simulink model "DPC_POWER_RAHMAN_original(1)"  (R2022a)
settings: Solver=VariableStepAuto  StartTime=0.0  StopTime=10  FixedStep=Ts  RelTol=1e-3
undefined symbols (not defined in the file): Ts
libraries: spsACVoltageSourceLib x2, spsSeriesRLCBranchLib x2, spsabctoAlphaBetaZeroLib x2, spsControlledVoltageSourceLib x1, spsCurrentMeasurementLib x1, spsGroundLib x1, spsThreePhaseSeriesRLCBranchLib x1, slpidlib x1, spsThreePhaseVIMeasurementLib x1, spsUniversalBridgeLib x1, spsVoltageMeasurementLib x1, spspowerguiLib x1
settings Model: Creator=ARAM  LastModifiedBy=Alireza Jabbarnejad
settings SolverCC: AlgebraicLoopSolver=TrustRegion
settings DataIOCC: ReturnWorkspaceOutputs=off
settings OptimizationCC: LifeSpan=inf
settings DebuggingCC: UnconnectedInputMsg=warning  UnconnectedOutputMsg=warning  UnconnectedLineMsg=warning  SFMachineParentedDataDiag=warning  ArithmeticOperatorsInVariantConditions=warning
settings SFSimCC: SimUseLocalCustomCode=off  CustomCodeUndefinedFunction=UseInterfaceOnly
settings RTWCC: RTWUseLocalCustomCode=off  DLArmComputeVersion=19.05
settings CodeAppCC: StateflowObjectComments=on
settings SimscapeCC: SimscapeNormalizeSystem=off

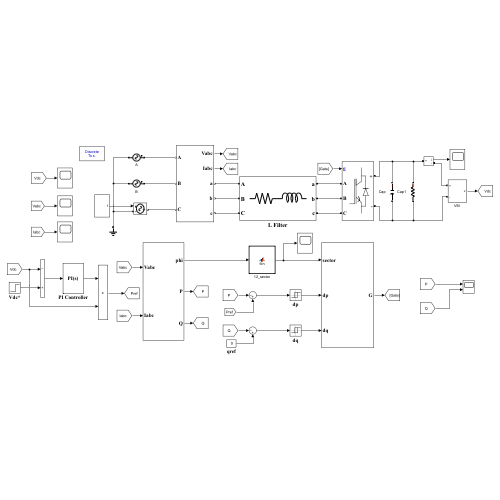
[thumbnail: Simulink's stored preview of the top-level diagram]
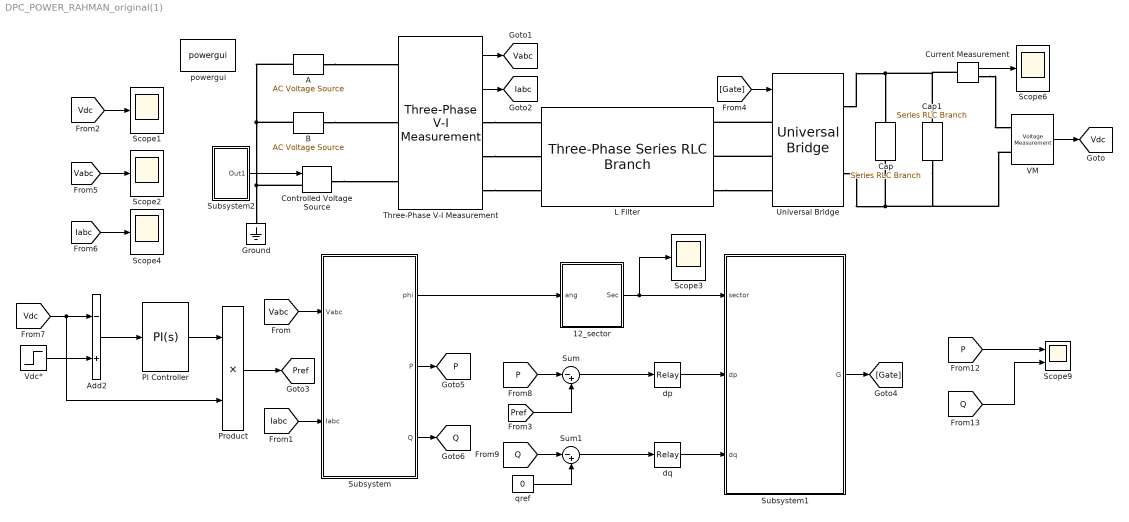
== system DPC_POWER_RAHMAN_original(1) ==
  12_sector : MATLAB Function  TreatAsAtomicUnit=on
  "A " : spsACVoltageSourceLib/AC Voltage Source  Amplitude=e*sqrt(2)  Phase=0  Frequency=50  SampleTime=0  Measurements=None  BusType=swing  Pref=10e3  Qref=0  Qmin=-inf  Qmax=+inf
  Add2 : Sum  Inputs=-+
  B : spsACVoltageSourceLib/AC Voltage Source  Amplitude=e*sqrt(2)  Phase=-120  Frequency=50  SampleTime=0  Measurements=None  BusType=swing  Pref=10e3  Qref=0  Qmin=-inf  Qmax=+inf
  Cap : spsSeriesRLCBranchLib/Series RLC Branch  LConnTagsString=__new0  RConnTagsString=__new0  BranchType=C  Resistance=1  Inductance=1e-3  SetiL0=off  InitialCurrent=0  Capacitance=10.8e-3  Setx0=on  InitialVoltage=150  Measurements=None
  Cap1 : spsSeriesRLCBranchLib/Series RLC Branch  LConnTagsString=__new0  RConnTagsString=__new0  BranchType=R  Resistance=57  Inductance=1e-3  SetiL0=off  InitialCurrent=0  Capacitance=2000e-6  Setx0=off  InitialVoltage=0  Measurements=None
  Controlled Voltage Source : spsControlledVoltageSourceLib/Controlled Voltage Source  Initialize=on  Source_Type=AC  Amplitude=150*sqrt(2)/sqrt(3)  Phase=120  Frequency=60  Measurements=None
  Current Measurement : spsCurrentMeasurementLib/Current Measurement  PhasorSimulation=off  OutputType=Complex  PSBequivalent=0
  Ground : spsGroundLib/Ground  LConnTagsString=a
  L Filter : spsThreePhaseSeriesRLCBranchLib/Three-Phase Series RLC Branch  LConnTagsString=A|B|C  RConnTagsString=A|B|C  BranchType=RL  Resistance=.2  Inductance=15e-3  Capacitance=1e-6  Measurements=None
  PI Controller : slpidlib/PID Controller  Controller=PI  Form=Parallel  TimeDomain=Continuous-time  UseExternalTs=off  SampleTime=-1  IntegratorMethod=Forward Euler  FilterMethod=Forward Euler  ControllerParametersSource=internal  P=0.27  I=3  UseKiTs=off  D=0  N=100  UseFilter=on  TunerSelectOption=Transfer Function Based (PID Tuner App)  InitialConditionSource=internal  InitialConditionForIntegrator=0  InitialConditionForFilter=0  DifferentiatorICPrevScaledInput=0  ExternalReset=none  TrackingMode=off  Kt=1  LimitOutput=off  SatLimitsSource=internal  UpperSaturationLimit=inf  LowerSaturationLimit=-inf  LinearizeAsGain=on  AntiWindupMode=none  Kb=1  POutMin=[]  POutMax=[]  IOutMin=[]  IOutMax=[]  DOutMin=[]  DOutMax=[]  NOutMin=[]  NOutMax=[]  SumOutMin=[]  SumOutMax=[]  SaturationOutMin=[]  SaturationOutMax=[]  PParamMin=[]  PParamMax=[]  IParamMin=[]  IParamMax=[]  DParamMin=[]  DParamMax=[]  NParamMin=[]  NParamMax=[]  KbParamMin=[]  KbParamMax=[]  KtParamMin=[]  KtParamMax=[]  KbOutMin=[]  KbOutMax=[]  KtOutMin=[]  KtOutMax=[]  IntegratorOutMin=[]  IntegratorOutMax=[]  FilterOutMin=[]  FilterOutMax=[]  SumI1OutMin=[]  SumI1OutMax=[]  SumI2OutMin=[]  SumI2OutMax=[]  SumI3OutMin=[]  SumI3OutMax=[]  SumI4OutMin=[]  SumI4OutMax=[]  SumDOutMin=[]  SumDOutMax=[]  DifferentiatorOutMin=[]  DifferentiatorOutMax=[]  FilterDiffOutCoefMin=[]  FilterDiffOutCoefMax=[]  ReciprocalOutMin=[]  ReciprocalOutMax=[]  SumDenOutMin=[]  SumDenOutMax=[]  SumNumOutMin=[]  SumNumOutMax=[]  DivideOutMin=[]  DivideOutMax=[]  UdiffTsProdOutMin=[]  UdiffTsProdOutMax=[]  NTsProdOutMin=[]  NTsProdOutMax=[]  UintegralTsProdOutMin=[]  UintegralTsProdOutMax=[]  UngainTsProdOutMin=[]  UngainTsProdOutMax=[]  IntegratorContinuousStateAttributes=''  IntegratorStateMustResolveToSignalObject=off  IntegratorRTWStateStorageClass=Auto  FilterContinuousStateAttributes=''  FilterStateMustResolveToSignalObject=off  FilterRTWStateStorageClass=Auto  ParallelPVariant=InternalParameters  IdealPVariant=Disabled  IVariant=InternalParameters  DVariant=Disabled  IntegratorVariant=Continuous  SatVariant=Disabled  AWVariant=Passthrough  PCopyVariant=Disabled  TRVariant=Disabled  FdbkBlocksVariant=Forward  IdealPFdbkVariant=Disabled  SatFdbkVariant=Disabled  DerivativeFilterVariant=Disabled  NVariant=Disabled  NCopyVariant=Disabled_SignalSpec  FilterICVariant=Disabled  IntegratorICVariant=InternalICs  ExternalResetVariant=Disabled  TRSumVariant=Passthrough  SumFdbkVariant=Disabled  SumVariant=Sum_PI  TsampFilterVariant=InternalTs  TsampNgainVariant=Passthrough  TsampIntegralVariant=Passthrough  ExternalSaturationOutDataTypeStr=Inherit: Same as second input  aMode=0
  Product : Product
  Scope{1..4,6} (5 alike) : Scope
  Scope9 : Scope  NumInputPorts=2
  Subsystem : Subsystem
  Subsystem1 : Subsystem
  Subsystem2 : Subsystem
  Sum : Sum  Inputs=|-+
  Sum1 : Sum  Inputs=|-+
  Three-Phase V-I Measurement : spsThreePhaseVIMeasurementLib/Three-Phase V-I Measurement  VoltageMeasurement=phase-to-ground  SetLabelV=off  LabelV=Vabc  Vpu=off  VpuLL=off  CurrentMeasurement=yes  SetLabelI=off  LabelI=Iabc  Ipu=off  Pbase=100e6  Vbase=500e3  OutputType=Complex  PhasorSimulation=off  PSBequivalent=0
  Universal Bridge : spsUniversalBridgeLib/Universal Bridge  Arms=3  SnubberResistance=1e5  SnubberCapacitance=inf  Device=IGBT / Diodes  Ron=1e-3  Lon=0  ForwardVoltages="[  0  0  ]"  ForwardVoltage=0  GTOparameters=[ 10e-6 , 20e-6 ]  IGBTparameters=[ 1e-6 , 2e-6 ]  Measurements=None  Measurements_2=None  converterType=Rectifier
  "VM " : spsVoltageMeasurementLib/Voltage Measurement  PhasorSimulation=off  OutputType=Complex  PSBequivalent=0
  Vdc* : Step  Time=0  After=150  SampleTime=0
  dp : Relay  OnSwitchValue=1  OffSwitchValue=-1
  dq : Relay  OnSwitchValue=1  OffSwitchValue=-1
  powergui : spspowerguiLib/powergui  Priority=1  SimulationMode=Discrete  SampleTime=Ts  frequency=60  Iterations=50  frequencyindice=60  Pbase=100e6  ErrMax=1e-4  UnitsV=kV  UnitsW=MW  buscounter=0  FunctionMessages=off  echomessages=off  EnableUseOfTLC=off  CurrentSourceSwitches=off  DisableSnubberDevices=off  DisableRonSwitches=off  DisableVfSwitches=off  DisplayEquations=off  AutomaticDiscreteSolvers=off  SolverType=Tustin/Backward Euler (TBE)  Interpol=off  ExternalGateDelay=off  methode=off  Ts=10  x0status=blocks  SPID=off  SwTol=0  HookPort=off  NonlinearTolerance=1e-4  nMaxIteration=100  ContinueOnMaxIteration=off  RestoreLinks=warning  ResistiveCurrentMeasurement=off  Frange=[0:2:500]  Ylog=off  Xlog=on  ShowGrid=off  save=off  variable=ZData  structure=Iabc  ZoomFFT=off  StartTime=1  cycles=5  DisplayStyle=1  fundamental=60  FreqAxis=off  MaxFrequency=1000  frequencyindicesteady=1  RmsSteady=1  display=off
  qref : Constant  Value=0
  tag scope: Iabc=global, P=global, Pref=global, Q=global, Vabc=global, Vdc=global
  wires:
  "VM "/1 -> [Vdc]
  [Iabc] -> Subsystem/2(Iabc)
  12_sector/1(Sec) -> Scope3/1, Subsystem1/1(sector)
  dp/1 -> Subsystem1/2(dp)
  dq/1 -> Subsystem1/3(dq)
  Subsystem1/1(G) -> [Gate]
  [Vdc] -> Scope1/1
  [Iabc] -> Scope4/1
  [Vabc] -> Scope2/1
  Vdc*/1 -> Add2/2
  Add2/1 -> PI Controller/1
  [Gate] -> Universal Bridge/1
  [Vdc] -> Product/2, Add2/1
  PI Controller/1 -> Product/1
  Subsystem/2(P) -> [P]
  Sum/1 -> dp/1
  qref/1 -> Sum1/2
  Sum1/1 -> dq/1
  Subsystem2/1(Out1) -> Controlled Voltage Source/1
  Current Measurement/1 -> Scope6/1
  Subsystem/3(Q) -> [Q]
  [P] -> Scope9/1
  [Q] -> Scope9/2
  [Vabc] -> Subsystem/1(Vabc)
  Subsystem/1(phi) -> 12_sector/1(ang)
  Product/1 -> [Pref]
  [Pref] -> Sum/2
  Three-Phase V-I Measurement/1 -> [Vabc]
  Three-Phase V-I Measurement/2 -> [Iabc]
  [P] -> Sum/1
  [Q] -> Sum1/1
  connections:
  "A "/RConn1 -- Three-Phase V-I Measurement/LConn1
  B/RConn1 -- Three-Phase V-I Measurement/LConn2
  "A "/LConn1 -- B/LConn1 -- Controlled Voltage Source/LConn1 -- Ground/LConn1
  Three-Phase V-I Measurement/RConn1 -- L Filter/LConn1
  Three-Phase V-I Measurement/RConn2 -- L Filter/LConn2
  Three-Phase V-I Measurement/RConn3 -- L Filter/LConn3
  Universal Bridge/LConn1 -- L Filter/RConn1
  Universal Bridge/LConn2 -- L Filter/RConn2
  Universal Bridge/RConn2 -- "VM "/LConn2 -- Cap1/RConn1 -- Cap/RConn1
  Universal Bridge/RConn1 -- Current Measurement/LConn1 -- Cap1/LConn1 -- Cap/LConn1
  L Filter/RConn3 -- Universal Bridge/LConn3
  Controlled Voltage Source/RConn1 -- Three-Phase V-I Measurement/LConn3
  Current Measurement/RConn1 -- "VM "/LConn1

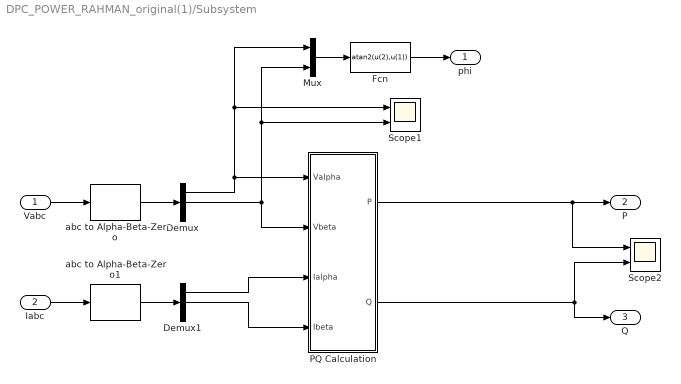
== system DPC_POWER_RAHMAN_original(1)/Subsystem ==
  Vabc : Inport
  Iabc : Inport  Port=2
  Demux : Demux  Outputs=3
  Demux1 : Demux  Outputs=3
  Fcn : Fcn  Expr=atan2(u(2),u(1))
  Mux : Mux  Inputs=2
  PQ Calculation : Subsystem
  Scope1 : Scope  NumInputPorts=2
  Scope2 : Scope  NumInputPorts=2
  abc to Alpha-Beta-Zero : spsabctoAlphaBetaZeroLib/abc to Alpha-Beta-Zero
      settings: SourceProductBaseCode=PS
  abc to Alpha-Beta-Zero1 : spsabctoAlphaBetaZeroLib/abc to Alpha-Beta-Zero
      settings: SourceProductBaseCode=PS
  phi : Outport
  P : Outport  Port=2
  Q : Outport  Port=3
  wires:
  PQ Calculation/1(P) -> P/1, Scope2/1
  PQ Calculation/2(Q) -> Scope2/2, Q/1
  Fcn/1 -> phi/1
  Mux/1 -> Fcn/1
  Vabc/1 -> abc to Alpha-Beta-Zero/1
  Demux/2 -> PQ Calculation/2(Vbeta), Mux/2, Scope1/2
  Demux1/1 -> PQ Calculation/3(Ialpha)
  Demux1/2 -> PQ Calculation/4(Ibeta)
  Demux/1 -> Mux/1, Scope1/1, PQ Calculation/1(Valpha)
  Iabc/1 -> abc to Alpha-Beta-Zero1/1
  abc to Alpha-Beta-Zero/1 -> Demux/1
  abc to Alpha-Beta-Zero1/1 -> Demux1/1

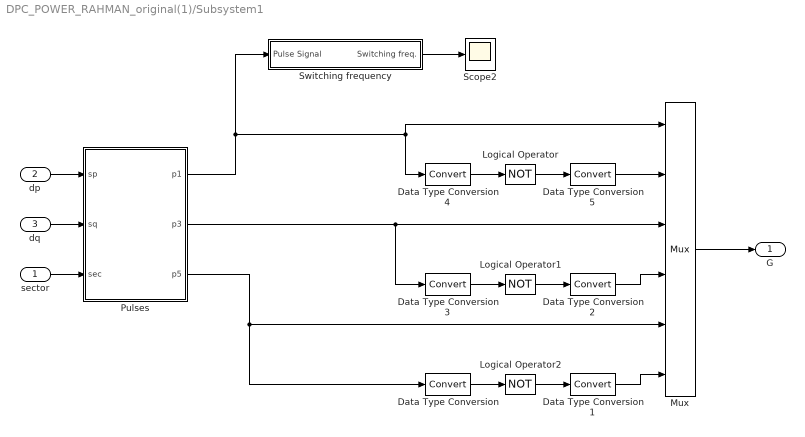
== system DPC_POWER_RAHMAN_original(1)/Subsystem1 ==
  sector : Inport
  dp : Inport  Port=2
  dq : Inport  Port=3
  " Pulses" : MATLAB Function  TreatAsAtomicUnit=on
  Data Type Conversion{,1..5} (6 alike) : DataTypeConversion
  Logical Operator : Logic  Operator=NOT
  Logical Operator1 : Logic  Operator=NOT
  Logical Operator2 : Logic  Operator=NOT
  Mux : Mux  Inputs=6
  Scope2 : Scope
  "Switching frequency " : Subsystem
  G : Outport
  wires:
  Logical Operator2/1 -> Data Type Conversion1/1
  Logical Operator1/1 -> Data Type Conversion2/1
  Logical Operator/1 -> Data Type Conversion5/1
  " Pulses"/2(p3) -> Data Type Conversion3/1, Mux/3
  " Pulses"/1(p1) -> Data Type Conversion4/1, Mux/1, "Switching frequency "/1(Pulse Signal)
  Mux/1 -> G/1
  Data Type Conversion/1 -> Logical Operator2/1
  Data Type Conversion1/1 -> Mux/6
  Data Type Conversion2/1 -> Mux/4
  Data Type Conversion3/1 -> Logical Operator1/1
  Data Type Conversion4/1 -> Logical Operator/1
  Data Type Conversion5/1 -> Mux/2
  " Pulses"/3(p5) -> Data Type Conversion/1, Mux/5
  "Switching frequency "/1(Switching freq.) -> Scope2/1
  sector/1 -> " Pulses"/3(sec)
  dq/1 -> " Pulses"/2(sq)
  dp/1 -> " Pulses"/1(sp)

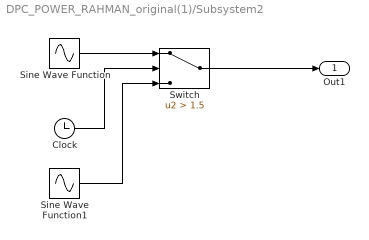
== system DPC_POWER_RAHMAN_original(1)/Subsystem2 ==
  Clock : Clock
  Sine Wave Function : Sin  Amplitude=e*sqrt(2)  Frequency=2*pi*50  Phase=2*pi/3  SampleTime=5e-6
  Sine Wave Function1 : Sin  Amplitude=e*sqrt(2)  Frequency=2*pi*50  Phase=2*pi/3  SampleTime=5e-6
  Switch : Switch  Criteria=u2 > Threshold  Threshold=1.5  SaturateOnIntegerOverflow=off  InputSameDT=off
  Out1 : Outport
  wires:
  Switch/1 -> Out1/1
  Sine Wave Function1/1 -> Switch/3
  Clock/1 -> Switch/2
  Sine Wave Function/1 -> Switch/1

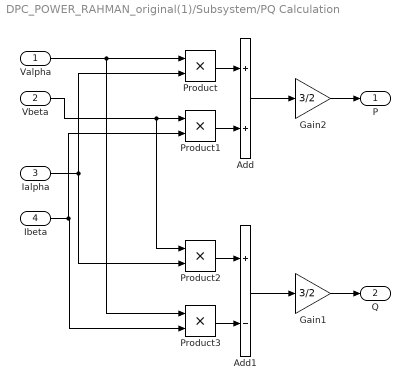
== system DPC_POWER_RAHMAN_original(1)/Subsystem/PQ Calculation ==
  Valpha : Inport
  Vbeta : Inport  Port=2
  Ialpha : Inport  Port=3
  Ibeta : Inport  Port=4
  Add : Sum
  Add1 : Sum  Inputs=+-
  Gain1 : Gain  Gain=3/2
  Gain2 : Gain  Gain=3/2
  Product{,1..3} (4 alike) : Product
  P : Outport
  Q : Outport  Port=2
  wires:
  Product1/1 -> Add/2
  Valpha/1 -> Product/1, Product3/1
  Product3/1 -> Add1/2
  Product2/1 -> Add1/1
  Add1/1 -> Gain1/1
  Add/1 -> Gain2/1
  Product/1 -> Add/1
  Ibeta/1 -> Product1/2, Product3/2
  Ialpha/1 -> Product/2, Product2/2
  Vbeta/1 -> Product2/1, Product1/1
  Gain2/1 -> P/1
  Gain1/1 -> Q/1

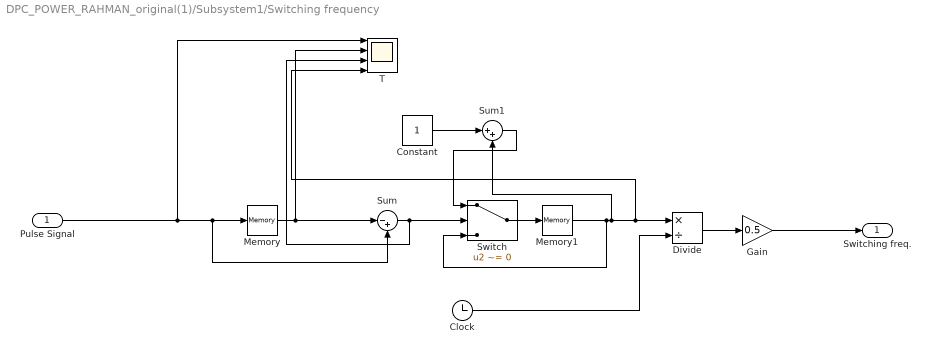
== system DPC_POWER_RAHMAN_original(1)/Subsystem1/Switching frequency  ==
  Pulse Signal : Inport
  Clock : Clock
  Constant : Constant
  Divide : Product  Inputs=*/
  Gain : Gain  Gain=0.5
  Memory : Memory
  Memory1 : Memory
  Sum : Sum  Inputs=|-+
  Sum1 : Sum  Inputs=|++
  Switch : Switch  Criteria=u2 ~= 0  SaturateOnIntegerOverflow=off  InputSameDT=off
  T : Scope  NumInputPorts=4
  Switching freq. : Outport
  wires:
  Gain/1 -> Switching freq./1
  Clock/1 -> Divide/2
  Divide/1 -> Gain/1
  Pulse Signal/1 -> Memory/1, Sum/2, T/1
  Sum1/1 -> Switch/1
  Memory/1 -> Sum/1, T/2
  Sum/1 -> Switch/2, T/3
  Constant/1 -> Sum1/1
  Switch/1 -> Memory1/1
  Memory1/1 -> Switch/3, Sum1/2, Divide/1, T/4

== matlab function DPC_POWER_RAHMAN_original(1)/Subsystem1/ Pulses ==
  data: sp input; p1 output; sq input; sec input; p3 output; p5 output
function [p1,p3,p5] = fcn(sp,sq,sec)
%#codegen
% % format of the array sw_array(x,z)

sw_array=zeros(3,12);  % initialize the switching table
% % x=[legA Leg B LegC]  % Z=[sector1 sector2 ..]
if((sp==1)&&(sq==0))
    
sw_array(:,1)=[1;0;1]; %sector 1
sw_array(:,2)=[1;0;1]; %sector 2
sw_array(:,3)=[1;0;0]; %sector 3
sw_array(:,4)=[1;0;0]; %sector 4
sw_array(:,5)=[1;1;0]; %sector 5
sw_array(:,6)=[1;1;0]; %sector 6
sw_array(:,7)=[0;1;0]; %sector 7
sw_array(:,8)=[0;1;0]; %sector 8
sw_array(:,9)=[0;1;1]; %sector 9
sw_array(:,10)=[0;1;1];%sector 10
sw_array(:,11)=[0;0;1]; %sector 11
sw_array(:,12)=[0;0;1]; %sector 12
 
elseif((sp==1)&&(sq==1))
sw_array(:,1)=[0;1;1]; %sector 1
sw_array(:,2)=[0;1;1]; %sector 2
sw_array(:,3)=[0;0;1]; %sector 3
sw_array(:,4)=[0;0;1]; %sector 4
sw_array(:,5)=[1;0;1]; %sector 5
sw_array(:,6)=[1;0;1]; %sector 6
sw_array(:,7)=[1;0;0]; %sector 7
sw_array(:,8)=[1;0;0]; %sector 8
sw_array(:,9)=[1;1;0]; %sector 9
sw_array(:,10)=[1;1;0]; %sector 10
sw_array(:,11)=[0;1;0]; %sector 11
sw_array(:,12)=[0;1;0]; %sector 12
 

elseif((sp==0)&&(sq==0))
sw_array(:,1)=[1;0;0]; %sector 1
sw_array(:,2)=[1;0;0]; %sector 2
sw_array(:,3)=[1;1;0]; %sector 3
sw_array(:,4)=[1;1;0]; %sector 4
sw_array(:,5)=[0;1;0]; %sector 5
sw_array(:,6)=[0;1;0]; %sector 6
sw_array(:,7)=[0;1;1]; %sector 7
sw_array(:,8)=[0;1;1]; %sector 8
sw_array(:,9)=[0;0;1]; %sector 9
sw_array(:,10)=[0;0;1]; %sector 10
sw_array(:,11)=[1;0;1]; %sector 11
sw_array(:,12)=[1;0;1]; %sector 12
 
elseif((sp==0)&&(sq==1))
sw_array(:,1)=[1;1;0]; %sector 1
sw_array(:,2)=[1;1;0]; %sector 2
sw_array(:,3)=[0;1;0]; %sector 3
sw_array(:,4)=[0;1;0]; %sector 4
sw_array(:,5)=[0;1;1]; %sector 5
sw_array(:,6)=[0;1;1]; %sector 6
sw_array(:,7)=[0;0;1]; %sector 7
sw_array(:,8)=[0;0;1]; %sector 8
sw_array(:,9)=[1;0;1]; %sector 9
sw_array(:,10)=[1;0;1]; %sector 10
sw_array(:,11)=[1;0;0]; %sector 11
sw_array(:,12)=[1;0;0]; %sector 12
end

p1=sw_array(1,sec);

p3=sw_array(2,sec);

p5=sw_array(3,sec);

% Merged Pulse






end

== matlab function DPC_POWER_RAHMAN_original(1)/12_sector ==
  data: ang input; Sec output
function Sec  = fcn(ang)
%convert to polar format



alpha=ang*180/pi;

% Sector calculation
Sec = (alpha>0 & alpha<=30)*1+ (alpha>30 & alpha<=60)*2+(alpha>60 & alpha<=90)*3  +(alpha>90 & alpha<=120)*4+ (alpha>120 & alpha<=150)*5  + (alpha>150 & alpha<=180)*6 ...
  +(alpha>=-180 & alpha<-150)*7+ (alpha>-150 & alpha<=-120)*8 + (alpha>-120 & alpha<=-90)*9 + +(alpha>-90 & alpha<-60)*10+ (alpha>-60 & alpha<=-30)*11 + (alpha>-30 & alpha<=0)*12;


%  determine whether sector is an odd number
% odd_sec=mod(floor(Sec),2);
